simulink subsystem "adaptiveEcm"  (R2025b)
settings: Solver=VariableStepAuto  StartTime=0.0  StopTime=10.0  RelTol=1e-3
values from neighbouring files (symbols this model uses):
  ECM = ecmParams(TempDep=false, Degradation=false, IC=struct("soc0", zD(1, :), "T0C", mean(tC(1, :))))    [checkFastPlant.m]
undefined symbols (not defined in the file or in its folder): diff, trace
(part 1 of 2)
settings Model: Creator=SC-Br  LastModifiedBy=SC-Br

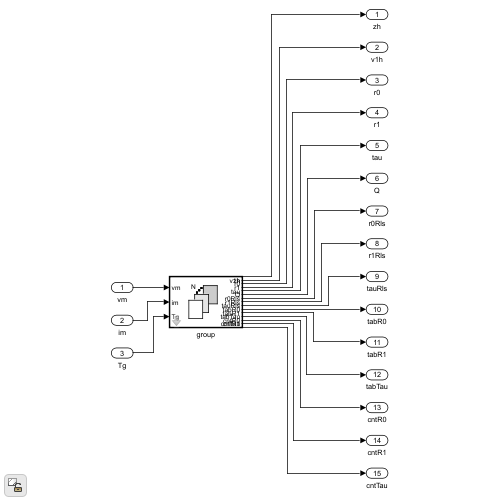
[thumbnail: Simulink's stored preview of the top-level diagram]
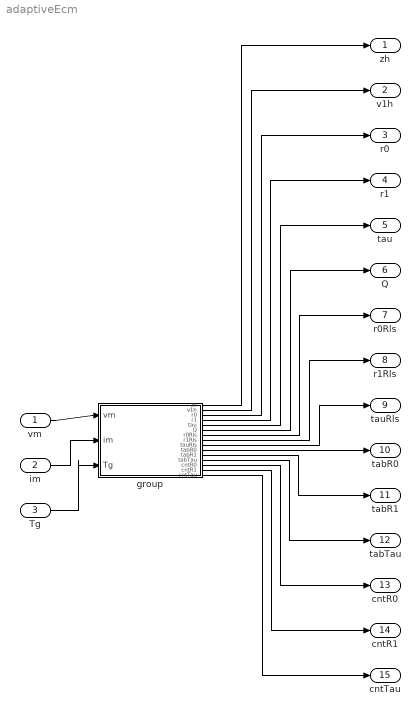
== system adaptiveEcm ==
  vm : Inport
  im : Inport  Port=2
  Tg : Inport  Port=3
  group : Subsystem  TreatAsAtomicUnit=on  mask{r0Init=ECM.est.init.r0, r1Init=ECM.est.init.r1, tauInit=ECM.est.init.tau, c0Init=ECM.est.init.count(:,:,:,1), c1Init=ECM.est.init.count(:,:,:,2), c2Init=ECM.est.init.count(:,:,:,3), QInit=ECM.est.init.Q, th0Init=ECM.est.init.th0, thRcInit=ECM.est.init.thRc, phiInit=ECM.est.init.phi}
  zh : Outport
  v1h : Outport  Port=2
  r0 : Outport  Port=3
  r1 : Outport  Port=4
  tau : Outport  Port=5
  Q : Outport  Port=6
  r0Rls : Outport  Port=7
  r1Rls : Outport  Port=8
  tauRls : Outport  Port=9
  tabR0 : Outport  Port=10
  tabR1 : Outport  Port=11
  tabTau : Outport  Port=12
  cntR0 : Outport  Port=13
  cntR1 : Outport  Port=14
  cntTau : Outport  Port=15
  wires:
  Tg/1 -> group/3(Tg)
  vm/1 -> group/1(vm)
  im/1 -> group/2(im)
  group/5(tau) -> tau/1
  group/12(tabTau) -> tabTau/1
  group/4(r1) -> r1/1
  group/11(tabR1) -> tabR1/1
  group/3(r0) -> r0/1
  group/10(tabR0) -> tabR0/1
  group/2(v1h) -> v1h/1
  group/9(tauRls) -> tauRls/1
  group/1(zh) -> zh/1
  group/6(Q) -> Q/1
  group/7(r0Rls) -> r0Rls/1
  group/8(r1Rls) -> r1Rls/1
  group/13(cntR0) -> cntR0/1
  group/14(cntR1) -> cntR1/1
  group/15(cntTau) -> cntTau/1

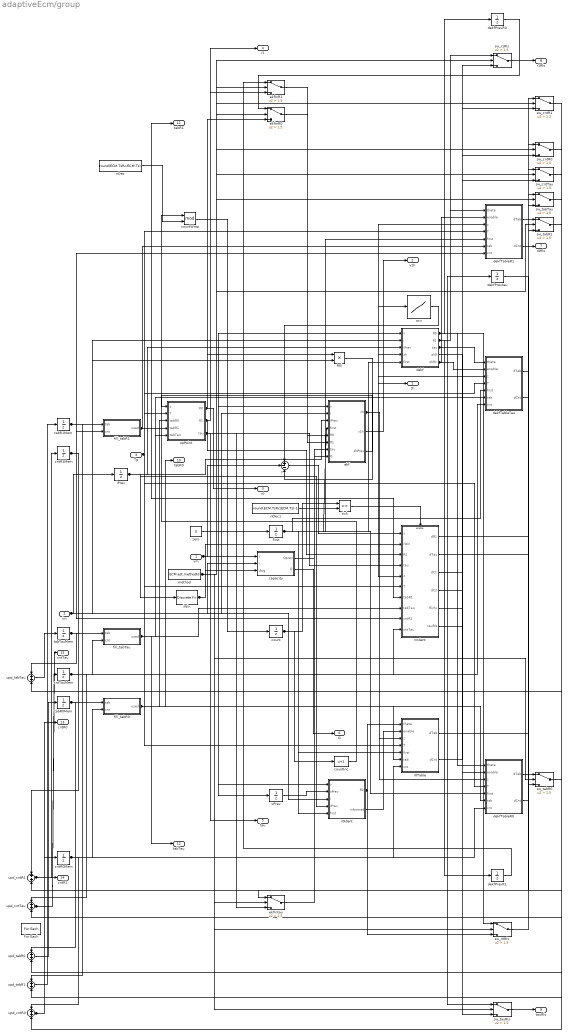
== system adaptiveEcm/group ==
  vm : Inport  PortDimensions=1  Partition=on  PartitionDimension=1  PartitionWidth=1  PartitionOffset=0
  im : Inport  Port=2  PortDimensions=1
  Tg : Inport  Port=3  PortDimensions=1  Partition=on  PartitionDimension=1  PartitionWidth=1  PartitionOffset=0
  For Each : ForEach  DisableCoverage=on  IterateSubsysMaskParameter=on,on,on,on,on,on,on,on,on,on  SubsysMaskParameterIterationDimension=3,3,3,3,3,3,2,2,2,2  SubsysMaskParameterIterationStepSize=1,1,1,1,1,1,1,1,1,1
  R0i : Product
  capacity : Subsystem
  cntR0Mem : UnitDelay  InitialCondition=c0Init  SampleTime=ECM.Ts  HasFrameUpgradeWarning=on
  cntR1Mem : UnitDelay  InitialCondition=c1Init  SampleTime=ECM.Ts  HasFrameUpgradeWarning=on
  cntTauMem : UnitDelay  InitialCondition=c2Init  SampleTime=ECM.Ts  HasFrameUpgradeWarning=on
  count : UnitDelay  SampleTime=ECM.Ts  HasFrameUpgradeWarning=on
  countInc : Bias  Bias=1  SaturateOnIntegerOverflow=off
  countWrap : Math  Operator=mod
  dekf : Subsystem
  dekfPrevR0 : UnitDelay  InitialCondition=exp(phiInit(1))  SampleTime=ECM.Ts  HasFrameUpgradeWarning=on
  dekfPrevR1 : UnitDelay  InitialCondition=exp(phiInit(2))  SampleTime=ECM.Ts  HasFrameUpgradeWarning=on
  dekfPrevtau : UnitDelay  InitialCondition=exp(phiInit(3))  SampleTime=ECM.Ts  HasFrameUpgradeWarning=on
  dekfTableR0 : Subsystem
  dekfTableR1 : Subsystem
  dekfTableTau : Subsystem
  ekf : Subsystem
  ekfInR0 : Switch  Criteria=u2 > Threshold  Threshold=1.5  SaturateOnIntegerOverflow=off  InputSameDT=off
  ekfInR1 : Switch  Criteria=u2 > Threshold  Threshold=1.5  SaturateOnIntegerOverflow=off  InputSameDT=off
  ekfIntau : Switch  Criteria=u2 > Threshold  Threshold=1.5  SaturateOnIntegerOverflow=off  InputSameDT=off
  fill_tabR0 : Subsystem
  fill_tabR1 : Subsystem
  fill_tabTau : Subsystem
  first : UnitDelay  InitialCondition=1  SampleTime=ECM.Ts  HasFrameUpgradeWarning=on
  iPrev : UnitDelay  SampleTime=ECM.Ts  HasFrameUpgradeWarning=on
  iWin : DiscreteFir  Coefficients=ones(1,round(ECM.TsRc/ECM.Ts))/round(ECM.TsRc/ECM.Ts)  SampleTime=ECM.Ts
  method : Constant  Value=ECM.est.methodId
  nDec : Constant  Value=round(ECM.TsRc/ECM.Ts)
  nDec1 : Constant  Value=round(ECM.TsRc/ECM.Ts)-1
  ocv : Lookup_n-D  NumberOfTableDimensions=1  BreakpointsForDimension1=ECM.est.socBp  Table=ECM.est.ocv  ExtrapMethod=Clip  UseLastTableValue=on  InternalRulePriority=Speed  RndMeth=Simplest
  opPoint : Subsystem
  r0Ident : Subsystem
  r0Table : Subsystem
  rcIdent : Subsystem  TreatAsAtomicUnit=on
  sw_cntR0 : Switch  Criteria=u2 > Threshold  Threshold=1.5  SaturateOnIntegerOverflow=off  InputSameDT=off
  sw_cntR1 : Switch  Criteria=u2 > Threshold  Threshold=1.5  SaturateOnIntegerOverflow=off  InputSameDT=off
  sw_cntTau : Switch  Criteria=u2 > Threshold  Threshold=1.5  SaturateOnIntegerOverflow=off  InputSameDT=off
  sw_r0Rls : Switch  Criteria=u2 > Threshold  Threshold=1.5  SaturateOnIntegerOverflow=off  InputSameDT=off
  sw_r1Rls : Switch  Criteria=u2 > Threshold  Threshold=1.5  SaturateOnIntegerOverflow=off  InputSameDT=off
  sw_tabR0 : Switch  Criteria=u2 > Threshold  Threshold=1.5  SaturateOnIntegerOverflow=off  InputSameDT=off
  sw_tabR1 : Switch  Criteria=u2 > Threshold  Threshold=1.5  SaturateOnIntegerOverflow=off  InputSameDT=off
  sw_tabTau : Switch  Criteria=u2 > Threshold  Threshold=1.5  SaturateOnIntegerOverflow=off  InputSameDT=off
  sw_tauRls : Switch  Criteria=u2 > Threshold  Threshold=1.5  SaturateOnIntegerOverflow=off  InputSameDT=off
  tabR0Mem : UnitDelay  InitialCondition=r0Init  SampleTime=ECM.Ts  HasFrameUpgradeWarning=on
  tabR1Mem : UnitDelay  InitialCondition=r1Init  SampleTime=ECM.Ts  HasFrameUpgradeWarning=on
  tabTauMem : UnitDelay  InitialCondition=tauInit  SampleTime=ECM.Ts  HasFrameUpgradeWarning=on
  tick : RelationalOperator  Operator===  OutDataTypeStr=boolean  RndMeth=Simplest  InputSameDT=off
  upd_cntR0 : Sum
  upd_cntR1 : Sum
  upd_cntTau : Sum
  upd_tabR0 : Sum
  upd_tabR1 : Sum
  upd_tabTau : Sum
  vPrev : UnitDelay  SampleTime=ECM.Ts  HasFrameUpgradeWarning=on
  y : Sum  Inputs=+--
  zero : Constant  Value=0
  zh : Outport  ConcatenationDimension=1
  v1h : Outport  Port=2  ConcatenationDimension=1
  r0 : Outport  Port=3  ConcatenationDimension=1
  r1 : Outport  Port=4  ConcatenationDimension=1
  tau : Outport  Port=5  ConcatenationDimension=1
  Q : Outport  Port=6  ConcatenationDimension=1
  r0Rls : Outport  Port=7  ConcatenationDimension=1
  r1Rls : Outport  Port=8  ConcatenationDimension=1
  tauRls : Outport  Port=9  ConcatenationDimension=1
  tabR0 : Outport  Port=10  ConcatenationDimension=3
  tabR1 : Outport  Port=11  ConcatenationDimension=3
  tabTau : Outport  Port=12  ConcatenationDimension=3
  cntR0 : Outport  Port=13  ConcatenationDimension=3
  cntR1 : Outport  Port=14  ConcatenationDimension=3
  cntTau : Outport  Port=15  ConcatenationDimension=3
  wires:
  upd_cntR0/1 -> cntR0Mem/1, cntR0/1
  tabR1Mem/1 -> upd_tabR1/1, fill_tabR1/1(tab)
  dekf/1(R0) -> dekfTableR0/1(theta), dekfPrevR0/1, sw_r0Rls/1
  fill_tabTau/1(used) -> dekfTableTau/6(tab), tabTau/1, rcIdent/8(tabTau), opPoint/5(tabTau)
  sw_tauRls/1 -> tauRls/1
  rcIdent/6(tauRls) -> sw_tauRls/3
  sw_r1Rls/1 -> r1Rls/1
  vm/1 -> ekf/1(v), r0Ident/1(v), dekf/1(v), vPrev/1, y/2, capacity/1(v)
  dekfPrevtau/1 -> ekfIntau/1
  zero/1 -> first/1
  nDec/1 -> countWrap/2
  sw_r0Rls/1 -> r0Rls/1
  r0Ident/2(informed) -> r0Table/2(enable)
  fill_tabR0/1(used) -> dekfTableR0/6(tab), r0Table/6(tab), opPoint/3(tabR0), tabR0/1
  dekfTableR1/1(dTab) -> sw_tabR1/1
  capacity/2(Q) -> Q/1
  rcIdent/5(R1rls) -> sw_r1Rls/3
  ekf/2(v1h) -> v1h/1
  fill_tabR1/1(used) -> dekfTableR1/6(tab), rcIdent/7(tabR1), opPoint/4(tabR1), tabR1/1
  ekfInR1/1 -> ekf/6(R1)
  rcIdent/4(dC2) -> sw_cntTau/3
  dekf/4(ok0) -> dekfTableR0/2(enable)
  dekfTableR0/1(dTab) -> sw_tabR0/1
  im/1 -> capacity/2(i), dekf/2(i), R0i/2, r0Ident/3(i), ekf/2(i), iPrev/1
  dekfTableTau/2(dCnt) -> sw_cntTau/1
  upd_tabR0/1 -> tabR0Mem/1
  opPoint/1(R0) -> R0i/1, ekfInR0/3, r0/1
  sw_tabTau/1 -> upd_tabTau/2
  ekf/3(zhPrev) -> opPoint/1(z)
  ekfInR0/1 -> ekf/5(R0)
  opPoint/2(R1) -> rcIdent/3(R1), r1/1, ekfInR1/3
  ekf/1(zh) -> dekfTableTau/3(z), dekfTableR1/3(z), dekfTableR0/3(z), ocv/1, rcIdent/5(z), dekf/4(zh), zh/1, r0Table/3(z)
  dekfTableTau/1(dTab) -> sw_tabTau/1
  cntR1Mem/1 -> upd_cntR1/1, rcIdent/9(cntR1), dekfTableR1/7(cnt), fill_tabR1/2(cnt)
  iWin/1 -> rcIdent/2(iWin), capacity/3(iAvg)
  dekfTableR1/2(dCnt) -> sw_cntR1/1
  rcIdent/3(dC1) -> sw_cntR1/3
  cntTauMem/1 -> upd_cntTau/1, rcIdent/10(cntTau), dekfTableTau/7(cnt), fill_tabTau/2(cnt)
  rcIdent/1(dR1) -> sw_tabR1/3
  r0Ident/1(R0) -> sw_r0Rls/3, r0Table/1(theta)
  first/1 -> dekfTableR1/5(first), dekfTableTau/5(first), dekfTableR0/5(first), dekf/5(first), r0Ident/5(first), r0Table/5(first), ekf/4(first)
  sw_tabR1/1 -> upd_tabR1/2
  opPoint/3(tau) -> rcIdent/4(tau), tau/1, ekfIntau/3
  dekfTableR0/2(dCnt) -> sw_cntR0/1
  countWrap/1 -> count/1
  dekf/3(tau) -> dekfTableTau/1(theta), sw_tauRls/1, dekfPrevtau/1
  upd_cntTau/1 -> cntTauMem/1, cntTau/1
  Tg/1 -> dekfTableR0/4(T), dekfTableTau/4(T), dekfTableR1/4(T), rcIdent/6(T), opPoint/2(T), r0Table/4(T)
  capacity/1(Qprev) -> ekf/8(Q)
  ekfIntau/1 -> ekf/7(tau)
  vPrev/1 -> r0Ident/2(vPrev)
  method/1 -> sw_tabR0/2, sw_tabR1/2, sw_cntR1/2, sw_tabTau/2, sw_r1Rls/2, sw_tauRls/2, sw_r0Rls/2, sw_cntTau/2, ekfInR1/2, ekfIntau/2, sw_cntR0/2, ekfInR0/2
  nDec1/1 -> tick/2
  iPrev/1 -> r0Ident/4(iPrev), ekf/3(iPrev), dekf/3(iPrev), iWin/1
  upd_tabTau/1 -> tabTauMem/1
  upd_cntR1/1 -> cntR1Mem/1, cntR1/1
  r0Table/1(dTab) -> sw_tabR0/3
  dekfPrevR0/1 -> ekfInR0/1
  upd_tabR1/1 -> tabR1Mem/1
  dekf/5(okRc) -> dekfTableR1/2(enable), dekfTableTau/2(enable)
  dekf/2(R1) -> dekfTableR1/1(theta), dekfPrevR1/1, sw_r1Rls/1
  count/1 -> countInc/1, tick/1
  tabTauMem/1 -> upd_tabTau/1, fill_tabTau/1(tab)
  cntR0Mem/1 -> upd_cntR0/1, r0Table/7(cnt), dekfTableR0/7(cnt), fill_tabR0/2(cnt)
  sw_cntR0/1 -> upd_cntR0/2
  tabR0Mem/1 -> upd_tabR0/1, fill_tabR0/1(tab)
  y/1 -> rcIdent/1(y)
  r0Table/2(dCnt) -> sw_cntR0/3
  rcIdent/2(dTau) -> sw_tabTau/3
  tick/1 -> rcIdent/Enable
  R0i/1 -> y/3
  countInc/1 -> countWrap/1
  sw_tabR0/1 -> upd_tabR0/2
  dekfPrevR1/1 -> ekfInR1/1
  ocv/1 -> y/1
  sw_cntR1/1 -> upd_cntR1/2
  sw_cntTau/1 -> upd_cntTau/2

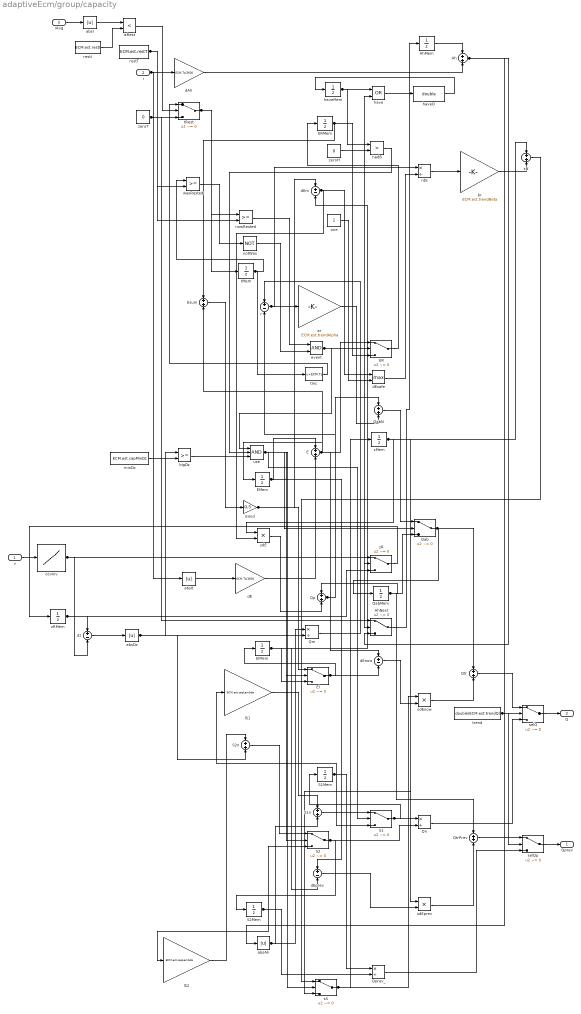
== system adaptiveEcm/group/capacity ==
  v : Inport  PortDimensions=1
  i : Inport  Port=2  PortDimensions=1
  iAvg : Inport  Port=3  PortDimensions=1
  Ah : Sum
  AhMem : UnitDelay  SampleTime=ECM.Ts  HasFrameUpgradeWarning=on
  AhNext : Switch  Criteria=u2 ~= 0  SaturateOnIntegerOverflow=off  InputSameDT=off
  E : Sum
  EMem : UnitDelay  SampleTime=ECM.Ts  HasFrameUpgradeWarning=on
  ER : Switch  Criteria=u2 ~= 0  SaturateOnIntegerOverflow=off  InputSameDT=off
  ERMem : UnitDelay  SampleTime=ECM.Ts  HasFrameUpgradeWarning=on
  El : Switch  Criteria=u2 ~= 0  SaturateOnIntegerOverflow=off  InputSameDT=off
  ElMem : UnitDelay  SampleTime=ECM.Ts  HasFrameUpgradeWarning=on
  Emid : Gain  Gain=0.5
  Esum : Sum
  Qab : Switch  Criteria=u2 ~= 0  SaturateOnIntegerOverflow=off  InputSameDT=off
  QabMem : UnitDelay  InitialCondition=QInit  SampleTime=ECM.Ts  HasFrameUpgradeWarning=on
  QabN : Sum
  Qm : Product  Inputs=*/
  Qn : Product  Inputs=*/
  Qp : Sum
  Qprev_ : Product  Inputs=*/
  Qtr : Sum
  QtrPrev : Sum
  S1 : Switch  Criteria=u2 ~= 0  SaturateOnIntegerOverflow=off  InputSameDT=off
  S1Mem : UnitDelay  InitialCondition=ECM.est.capW0*QInit  SampleTime=ECM.Ts  HasFrameUpgradeWarning=on
  S1n : Sum
  S2 : Switch  Criteria=u2 ~= 0  SaturateOnIntegerOverflow=off  InputSameDT=off
  S2Mem : UnitDelay  InitialCondition=ECM.est.capW0  SampleTime=ECM.Ts  HasFrameUpgradeWarning=on
  S2n : Sum
  absAh : Abs  SaturateOnIntegerOverflow=off
  absDz : Abs  SaturateOnIntegerOverflow=off
  absI : Abs  SaturateOnIntegerOverflow=off
  absIt : Abs  SaturateOnIntegerOverflow=off
  ar : Gain  Gain=ECM.est.trendAlpha
  bigDz : RelationalOperator  OutDataTypeStr=boolean  RndMeth=Simplest  InputSameDT=off
  br : Gain  Gain=ECM.est.trendBeta
  dAh : Gain  Gain=ECM.Ts/3600
  dE : Gain  Gain=ECM.Ts/3600
  dEm : Sum  Inputs=+-
  dEnow : Sum  Inputs=+-
  dEprev : Sum  Inputs=+-
  dEsafe : MinMax  Function=max  Inputs=2
  dz : Sum  Inputs=+-
  event : Logic  AllPortsSameDT=off  OutDataTypeStr=boolean
  hadB : RelationalOperator  Operator=>  OutDataTypeStr=boolean  RndMeth=Simplest  InputSameDT=off
  have : Logic  Operator=OR  AllPortsSameDT=off  OutDataTypeStr=boolean
  haveD : DataTypeConversion  OutDataTypeStr=double  SaturateOnIntegerOverflow=off  RndMeth=Floor
  haveMem : UnitDelay  SampleTime=ECM.Ts  HasFrameUpgradeWarning=on
  isRest : RelationalOperator  Operator=<  OutDataTypeStr=boolean  RndMeth=Simplest  InputSameDT=off
  lS1 : Gain  Gain=ECM.est.capLambda
  lS2 : Gain  Gain=ECM.est.capLambda
  minDz : Constant  Value=ECM.est.capMinDz
  notWas : Logic  Operator=NOT  AllPortsSameDT=off  OutDataTypeStr=boolean
  nowRested : RelationalOperator  OutDataTypeStr=boolean  RndMeth=Simplest  InputSameDT=off
  ocvInv : Lookup_n-D  NumberOfTableDimensions=1  BreakpointsForDimension1=ECM.est.ocv  Table=ECM.est.socBp  ExtrapMethod=Clip  UseLastTableValue=on  InternalRulePriority=Speed  RndMeth=Simplest
  one : Constant
  r : Sum  Inputs=+-
  rdE : Product  Inputs=*/
  restI : Constant  Value=ECM.est.restI
  restT : Constant  Value=ECM.est.restT
  sMem : UnitDelay  SampleTime=ECM.Ts  HasFrameUpgradeWarning=on
  sN : Sum
  sS : Switch  Criteria=u2 ~= 0  SaturateOnIntegerOverflow=off  InputSameDT=off
  sdE : Product
  sdEnow : Product
  sdEprev : Product
  selQ : Switch  Criteria=u2 ~= 0  SaturateOnIntegerOverflow=off  InputSameDT=off
  selQp : Switch  Criteria=u2 ~= 0  SaturateOnIntegerOverflow=off  InputSameDT=off
  tInc : Bias  Bias=ECM.Ts  SaturateOnIntegerOverflow=off
  tMem : UnitDelay  SampleTime=ECM.Ts  HasFrameUpgradeWarning=on
  tRest : Switch  Criteria=u2 ~= 0  SaturateOnIntegerOverflow=off  InputSameDT=off
  trend : Constant  Value=double(ECM.est.trendQ)
  use : Logic  Inputs=3  AllPortsSameDT=off  OutDataTypeStr=boolean
  wasRested : RelationalOperator  OutDataTypeStr=boolean  RndMeth=Simplest  InputSameDT=off
  zR : Switch  Criteria=u2 ~= 0  SaturateOnIntegerOverflow=off  InputSameDT=off
  zRMem : UnitDelay  SampleTime=ECM.Ts  HasFrameUpgradeWarning=on
  zeroH : Constant  Value=0
  zeroT : Constant  Value=0
  Qprev : Outport
  Q : Outport  Port=2
  wires:
  ERMem/1 -> Esum/1, ER/3
  absIt/1 -> dE/1
  v/1 -> ocvInv/1
  isRest/1 -> tRest/2
  ar/1 -> QabN/2
  wasRested/1 -> notWas/1
  restI/1 -> isRest/2
  event/1 -> use/1, have/2, AhNext/2, ER/2, zR/2
  iAvg/1 -> absI/1
  S2Mem/1 -> lS2/1, Qprev_/2, S2/3
  zRMem/1 -> dz/1, zR/3
  restT/1 -> nowRested/2, wasRested/2
  ocvInv/1 -> dz/2, zR/1
  absI/1 -> isRest/1
  dz/1 -> absDz/1
  i/1 -> absIt/1, dAh/1
  dEnow/1 -> sdEnow/2
  zeroT/1 -> AhNext/1, tRest/3
  nowRested/1 -> event/1
  minDz/1 -> bigDz/2
  absDz/1 -> Qm/2, S2n/2, bigDz/1
  dAh/1 -> Ah/2
  zR/1 -> zRMem/1
  tRest/1 -> tMem/1, nowRested/1
  one/1 -> dEsafe/2
  Esum/1 -> Emid/1
  bigDz/1 -> use/3
  lS2/1 -> S2n/1
  notWas/1 -> event/2
  zeroH/1 -> hadB/2
  tMem/1 -> tInc/1, wasRested/1
  r/1 -> rdE/1, ar/1
  use/1 -> S1/2, S2/2, Qab/2, El/2, sS/2
  tInc/1 -> tRest/1
  EMem/1 -> E/1, dEprev/1
  S2/1 -> S2Mem/1, Qn/2
  Emid/1 -> dEm/1, El/1
  sdE/1 -> Qp/2
  dE/1 -> E/2
  dEprev/1 -> sdEprev/2
  ElMem/1 -> dEm/2, El/3, dEprev/2
  lS1/1 -> S1n/1
  S2n/1 -> S2/1
  absAh/1 -> S1n/2, Qm/1
  haveMem/1 -> have/1, hadB/1
  dEm/1 -> sdE/2, dEsafe/1
  E/1 -> EMem/1, Esum/2, dEnow/1, ER/1
  dEsafe/1 -> rdE/2
  Qp/1 -> r/2, QabN/1
  AhMem/1 -> Ah/1
  have/1 -> haveD/1
  sS/1 -> sdEnow/1, sMem/1
  Qm/1 -> r/1
  El/1 -> ElMem/1, dEnow/2
  S1Mem/1 -> lS1/1, Qprev_/1, S1/3
  AhNext/1 -> AhMem/1
  Qprev_/1 -> selQp/3
  S1n/1 -> S1/1
  hadB/1 -> use/2
  ER/1 -> ERMem/1
  QabN/1 -> Qab/1
  sMem/1 -> sdE/1, sN/1, sdEprev/1, sS/3
  S1/1 -> S1Mem/1, Qn/1
  QabMem/1 -> Qp/1, QtrPrev/1, Qab/3
  haveD/1 -> haveMem/1
  rdE/1 -> br/1
  Qab/1 -> QabMem/1, Qtr/1
  sdEnow/1 -> Qtr/2
  Qn/1 -> selQ/3
  sdEprev/1 -> QtrPrev/2
  Ah/1 -> absAh/1, AhNext/3
  br/1 -> sN/2
  Qtr/1 -> selQ/1
  trend/1 -> selQ/2, selQp/2
  QtrPrev/1 -> selQp/1
  sN/1 -> sS/1
  selQ/1 -> Q/1
  selQp/1 -> Qprev/1

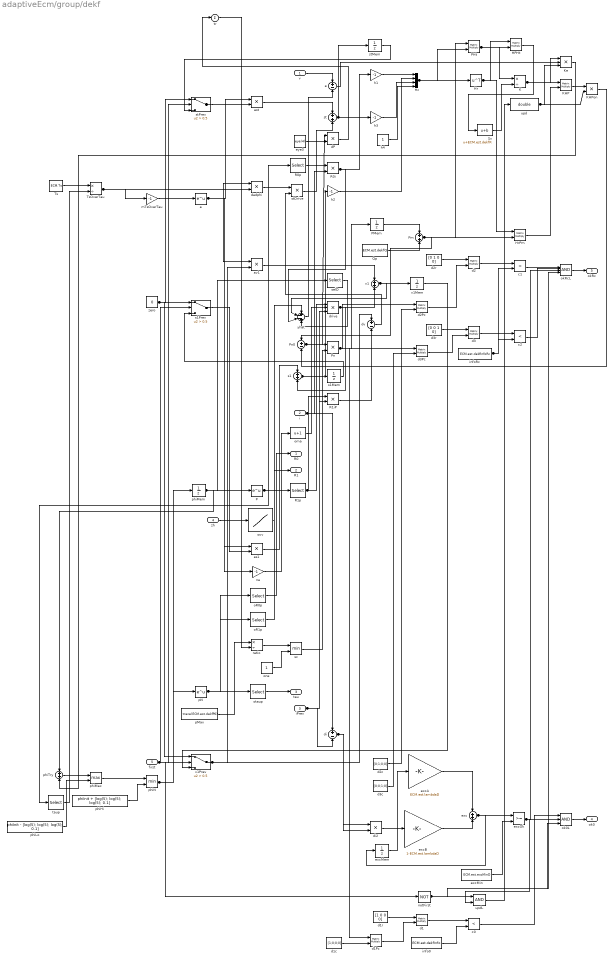
== system adaptiveEcm/group/dekf ==
  v : Inport  PortDimensions=1
  i : Inport  Port=2  PortDimensions=1
  iPrev : Inport  Port=3  PortDimensions=1
  zh : Inport  Port=4  PortDimensions=1
  first : Inport  Port=5  PortDimensions=1
  HPHt : Product  Multiplication=Matrix(*)
  Hc : Concatenate  NumInputs=4  Mode=Multidimensional array
  Hr : Math  Operator=transpose
  HrPm : Product  Multiplication=Matrix(*)
  K : Product  Inputs=*/
  KHP : Product  Multiplication=Matrix(*)
  KHPon : Product
  Ke : Product  Inputs=3
  PHt : Product  Multiplication=Matrix(*)
  PMem : UnitDelay  InitialCondition=ECM.est.dekfP0  SampleTime=ECM.Ts  HasFrameUpgradeWarning=on
  Pm : Sum
  Pn : Product
  Pn0 : Sum  Inputs=+-
  Qp : Constant  Value=ECM.est.dekfQ
  R0i : Product
  R0p : Selector  InputPortWidth=4  IndexOptions=Index vector (dialog)  Indices=1  OutputSizes=1
  R1iP : Product
  R1p : Selector  InputPortWidth=4  IndexOptions=Index vector (dialog)  Indices=2  OutputSizes=1
  Sv : Bias  Bias=ECM.est.dekfR  SaturateOnIntegerOverflow=off
  Ts : Constant  Value=ECM.Ts
  TsOverTau : Product  Inputs=*/
  a : Math
  as1 : Product
  ast : Product
  av1 : Product
  c0 : RelationalOperator  Operator=<  OutDataTypeStr=boolean  RndMeth=Simplest  InputSameDT=off
  c1 : RelationalOperator  Operator=<  OutDataTypeStr=boolean  RndMeth=Simplest  InputSameDT=off
  c2 : RelationalOperator  Operator=<  OutDataTypeStr=boolean  RndMeth=Simplest  InputSameDT=off
  d1 : Product  Multiplication=Matrix(*)
  d1Pc : Product  Multiplication=Matrix(*)
  d1c : Constant  Value=[1;0;0;0]  VectorParams1D=off
  d1r : Constant  Value=[1 0 0 0]  VectorParams1D=off
  d2 : Product  Multiplication=Matrix(*)
  d2Pc : Product  Multiplication=Matrix(*)
  d2c : Constant  Value=[0;1;0;0]  VectorParams1D=off
  d2r : Constant  Value=[0 1 0 0]  VectorParams1D=off
  d3 : Product  Multiplication=Matrix(*)
  d3Pc : Product  Multiplication=Matrix(*)
  d3c : Constant  Value=[0;0;1;0]  VectorParams1D=off
  d3r : Constant  Value=[0 0 1 0]  VectorParams1D=off
  dP : Product
  dadphi : Product
  di : Sum  Inputs=+-
  di2 : Product
  drive : Product  Inputs=3
  dv : Sum  Inputs=+-
  e : Sum  Inputs=+-
  exc : Sum
  excA : Gain  Gain=ECM.est.lambdaD
  excB : Gain  Gain=1-ECM.est.lambdaD
  excMem : UnitDelay  SampleTime=ECM.Ts  HasFrameUpgradeWarning=on
  excMin : Constant  Value=ECM.est.excMinD
  excOk : RelationalOperator  OutDataTypeStr=boolean  RndMeth=Simplest  InputSameDT=off
  eye3 : Constant  Value=eye(4)
  h1 : Gain  Gain=-1
  h2 : Gain  Gain=-1
  h3 : Gain  Gain=-1
  h4 : Constant
  info0 : Constant  Value=ECM.est.dekfInfo
  infoRc : Constant  Value=ECM.est.dekfInfoRc
  mTsOverTau : Gain  Gain=-1
  na : Gain  Gain=-1
  notFirst : Logic  Operator=NOT  AllPortsSameDT=off  OutDataTypeStr=boolean
  oR0p : Selector  InputPortWidth=4  IndexOptions=Index vector (dialog)  Indices=1  OutputSizes=1
  oR1p : Selector  InputPortWidth=4  IndexOptions=Index vector (dialog)  Indices=2  OutputSizes=1
  ocv : Lookup_n-D  NumberOfTableDimensions=1  BreakpointsForDimension1=ECM.est.socBp  Table=ECM.est.ocv  ExtrapMethod=Clip  UseLastTableValue=on  InternalRulePriority=Speed  RndMeth=Simplest
  ok0L : Logic  Inputs=3  AllPortsSameDT=off  OutDataTypeStr=boolean
  okRcL : Logic  Inputs=4  AllPortsSameDT=off  OutDataTypeStr=boolean
  oma : Bias  Bias=1  SaturateOnIntegerOverflow=off
  one : Constant
  otaup : Selector  InputPortWidth=4  IndexOptions=Index vector (dialog)  Indices=3  OutputSizes=1
  p : Math
  pMax : Constant  Value=trace(ECM.est.dekfP0)
  pN : Math
  phiHi : Constant  Value=phiInit + [log(5); log(5); log(5); 0.1]
  phiLo : Constant  Value=phiInit - [log(5); log(5); log(5); 0.1]
  phiMax : MinMax  Function=max  Inputs=2
  phiMem : UnitDelay  InitialCondition=phiInit  SampleTime=ECM.Ts  HasFrameUpgradeWarning=on
  phiN : MinMax  Inputs=2
  phiTry : Sum
  ratio : Product  Inputs=*/
  s1 : Sum
  s1Mem : UnitDelay  SampleTime=ECM.Ts  HasFrameUpgradeWarning=on
  s1Prev : Switch  Criteria=u2 > Threshold  Threshold=0.5  SaturateOnIntegerOverflow=off  InputSameDT=off
  sc : MinMax  Inputs=2
  selD : Selector  InputPortWidth=4  IndexOptions=Index vector (dialog)  Indices=4  OutputSizes=1
  st : Sum
  stDrive : Product
  stMem : UnitDelay  SampleTime=ECM.Ts  HasFrameUpgradeWarning=on
  stPrev : Switch  Criteria=u2 > Threshold  Threshold=0.5  SaturateOnIntegerOverflow=off  InputSameDT=off
  taup : Selector  InputPortWidth=4  IndexOptions=Index vector (dialog)  Indices=3  OutputSizes=1
  tr : Sum  Inputs=+
  upd : DataTypeConversion  OutDataTypeStr=double  SaturateOnIntegerOverflow=off  RndMeth=Floor
  updL : Logic  AllPortsSameDT=off  OutDataTypeStr=boolean
  v1 : Sum
  v1Mem : UnitDelay  SampleTime=ECM.Ts  HasFrameUpgradeWarning=on
  v1Prev : Switch  Criteria=u2 > Threshold  Threshold=0.5  SaturateOnIntegerOverflow=off  InputSameDT=off
  yhat : Sum  Inputs=+--+
  zero : Constant  Value=0
  R0 : Outport
  R1 : Outport  Port=2
  tau : Outport  Port=3
  ok0 : Outport  Port=4
  okRc : Outport  Port=5
  wires:
  selD/1 -> yhat/4
  TsOverTau/1 -> mTsOverTau/1, dadphi/2
  Hr/1 -> HPHt/1, HrPm/1
  dP/1 -> tr/1
  oma/1 -> drive/2
  R0p/1 -> R0i/1
  Pn0/1 -> dP/1, Pn/1
  pMax/1 -> ratio/1
  Ts/1 -> TsOverTau/1
  phiHi/1 -> phiN/2
  phiLo/1 -> phiMax/2
  stMem/1 -> stPrev/3
  phiTry/1 -> phiMax/1
  mTsOverTau/1 -> a/1
  sc/1 -> Pn/2
  h1/1 -> Hc/1
  v1Prev/1 -> dv/1, av1/2
  taup/1 -> TsOverTau/2
  iPrev/1 -> di/2, drive/3, R1iP/2
  phiMax/1 -> phiN/1
  R1p/1 -> drive/1, R1iP/1
  eye3/1 -> dP/2
  zero/1 -> v1Prev/1, s1Prev/1, stPrev/1
  e/1 -> Ke/2
  upd/1 -> KHPon/2, Ke/3
  first/1 -> v1Prev/2, s1Prev/2, stPrev/2, notFirst/1
  s1Mem/1 -> s1Prev/3
  R0i/1 -> yhat/3, h1/1
  phiN/1 -> phiMem/1, pN/1
  tr/1 -> ratio/2
  stPrev/1 -> ast/2
  s1Prev/1 -> as1/2
  a/1 -> av1/1, dadphi/1, na/1, ast/1, as1/1
  R1iP/1 -> dv/2
  phiMem/1 -> phiTry/1, selD/1, p/1
  zh/1 -> ocv/1
  pN/1 -> oR0p/1, otaup/1, oR1p/1
  ast/1 -> st/1
  stDrive/1 -> st/2
  dadphi/1 -> stDrive/1
  v1/1 -> yhat/2, v1Mem/1
  av1/1 -> v1/1
  h4/1 -> Hc/4
  p/1 -> taup/1, R0p/1, R1p/1
  di/1 -> di2/1, di2/2
  ocv/1 -> yhat/1
  yhat/1 -> e/2
  as1/1 -> s1/1
  na/1 -> oma/1
  oR0p/1 -> R0/1
  Pn/1 -> d3Pc/1, PMem/1, d1Pc/1, d2Pc/1
  drive/1 -> s1/2, v1/2
  oR1p/1 -> R1/1
  ratio/1 -> sc/1
  one/1 -> sc/2
  otaup/1 -> tau/1
  v/1 -> e/1
  s1/1 -> s1Mem/1, h2/1
  i/1 -> di/1, R0i/2
  st/1 -> stMem/1, h3/1
  h2/1 -> Hc/2
  d1c/1 -> d1Pc/2
  h3/1 -> Hc/3
  PMem/1 -> Pm/1
  Qp/1 -> Pm/2
  dv/1 -> stDrive/2
  d2c/1 -> d2Pc/2
  d3c/1 -> d3Pc/2
  di2/1 -> excB/1
  excMem/1 -> excA/1
  d1r/1 -> d1/1
  d1Pc/1 -> d1/2
  Hc/1 -> Hr/1, PHt/2
  Pm/1 -> Pn0/1, PHt/1, HrPm/2
  d2r/1 -> d2/1
  v1Mem/1 -> v1Prev/3
  d2Pc/1 -> d2/2
  d3r/1 -> d3/1
  d3Pc/1 -> d3/2
  excA/1 -> exc/1
  excB/1 -> exc/2
  notFirst/1 -> okRcL/4, updL/1, ok0L/3
  d1/1 -> c0/1
  info0/1 -> c0/2
  PHt/1 -> K/1, HPHt/2
  Sv/1 -> K/2
  d2/1 -> c1/1
  d3/1 -> c2/1
  infoRc/1 -> c1/2, c2/2
  exc/1 -> excOk/1, excMem/1
  excMin/1 -> excOk/2
  updL/1 -> upd/1
  c0/1 -> ok0L/1
  HPHt/1 -> Sv/1
  K/1 -> Ke/1, KHP/1
  HrPm/1 -> KHP/2
  c1/1 -> okRcL/1
  c2/1 -> okRcL/2
  excOk/1 -> updL/2, okRcL/3, ok0L/2
  Ke/1 -> phiTry/2
  KHP/1 -> KHPon/1
  okRcL/1 -> okRc/1
  ok0L/1 -> ok0/1
  KHPon/1 -> Pn0/2

== system adaptiveEcm/group/dekfTableR0 ==
  theta : Inport  PortDimensions=1
  enable : Inport  Port=2  PortDimensions=1
  z : Inport  Port=3  PortDimensions=1
  T : Inport  Port=4  PortDimensions=1
  first : Inport  Port=5  PortDimensions=1
  tab : Inport  Port=6  PortDimensions=[numel(ECM.est.socBp) numel(ECM.est.tBpC)]
  cnt : Inport  Port=7  PortDimensions=[numel(ECM.est.socBp) numel(ECM.est.tBpC)]
  TLag : Sum
  TLagA : Gain  Gain=ECM.est.lambdaD
  TLagB : Gain  Gain=1-ECM.est.lambdaD
  TLagMem : UnitDelay  SampleTime=-1  HasFrameUpgradeWarning=on
  TLagOld : Switch  Criteria=u2 > Threshold  Threshold=0.5  SaturateOnIntegerOverflow=off  InputSameDT=off
  nodeUpdate : Subsystem
  zLag : Sum
  zLagA : Gain  Gain=ECM.est.lambdaD
  zLagB : Gain  Gain=1-ECM.est.lambdaD
  zLagMem : UnitDelay  SampleTime=-1  HasFrameUpgradeWarning=on
  zLagOld : Switch  Criteria=u2 > Threshold  Threshold=0.5  SaturateOnIntegerOverflow=off  InputSameDT=off
  dTab : Outport
  dCnt : Outport  Port=2
  wires:
  z/1 -> zLagB/1, zLagOld/1
  TLagOld/1 -> TLagA/1
  TLagMem/1 -> TLagOld/3
  zLagA/1 -> zLag/1
  zLagB/1 -> zLag/2
  T/1 -> TLagOld/1, TLagB/1
  first/1 -> TLagOld/2, zLagOld/2
  zLagOld/1 -> zLagA/1
  TLag/1 -> TLagMem/1, nodeUpdate/4(T)
  TLagB/1 -> TLag/2
  TLagA/1 -> TLag/1
  theta/1 -> nodeUpdate/1(theta)
  zLag/1 -> zLagMem/1, nodeUpdate/3(z)
  enable/1 -> nodeUpdate/2(enable)
  zLagMem/1 -> zLagOld/3
  tab/1 -> nodeUpdate/5(tab)
  cnt/1 -> nodeUpdate/6(cnt)
  nodeUpdate/1(dTab) -> dTab/1
  nodeUpdate/2(dCnt) -> dCnt/1

== system adaptiveEcm/group/dekfTableR1 ==
  theta : Inport  PortDimensions=1
  enable : Inport  Port=2  PortDimensions=1
  z : Inport  Port=3  PortDimensions=1
  T : Inport  Port=4  PortDimensions=1
  first : Inport  Port=5  PortDimensions=1
  tab : Inport  Port=6  PortDimensions=[numel(ECM.est.socBp) numel(ECM.est.tBpC)]
  cnt : Inport  Port=7  PortDimensions=[numel(ECM.est.socBp) numel(ECM.est.tBpC)]
  TLag : Sum
  TLagA : Gain  Gain=ECM.est.lambdaD
  TLagB : Gain  Gain=1-ECM.est.lambdaD
  TLagMem : UnitDelay  SampleTime=-1  HasFrameUpgradeWarning=on
  TLagOld : Switch  Criteria=u2 > Threshold  Threshold=0.5  SaturateOnIntegerOverflow=off  InputSameDT=off
  nodeUpdate : Subsystem
  zLag : Sum
  zLagA : Gain  Gain=ECM.est.lambdaD
  zLagB : Gain  Gain=1-ECM.est.lambdaD
  zLagMem : UnitDelay  SampleTime=-1  HasFrameUpgradeWarning=on
  zLagOld : Switch  Criteria=u2 > Threshold  Threshold=0.5  SaturateOnIntegerOverflow=off  InputSameDT=off
  dTab : Outport
  dCnt : Outport  Port=2
  wires:
  z/1 -> zLagOld/1, zLagB/1
  first/1 -> zLagOld/2, TLagOld/2
  TLagOld/1 -> TLagA/1
  T/1 -> TLagB/1, TLagOld/1
  zLagA/1 -> zLag/1
  zLagB/1 -> zLag/2
  zLagOld/1 -> zLagA/1
  TLagA/1 -> TLag/1
  TLagB/1 -> TLag/2
  nodeUpdate/1(dTab) -> dTab/1
  theta/1 -> nodeUpdate/1(theta)
  zLag/1 -> zLagMem/1, nodeUpdate/3(z)
  enable/1 -> nodeUpdate/2(enable)
  tab/1 -> nodeUpdate/5(tab)
  TLag/1 -> nodeUpdate/4(T), TLagMem/1
  cnt/1 -> nodeUpdate/6(cnt)
  zLagMem/1 -> zLagOld/3
  nodeUpdate/2(dCnt) -> dCnt/1
  TLagMem/1 -> TLagOld/3

== system adaptiveEcm/group/dekfTableTau ==
  theta : Inport  PortDimensions=1
  enable : Inport  Port=2  PortDimensions=1
  z : Inport  Port=3  PortDimensions=1
  T : Inport  Port=4  PortDimensions=1
  first : Inport  Port=5  PortDimensions=1
  tab : Inport  Port=6  PortDimensions=[numel(ECM.est.socBp) numel(ECM.est.tBpC)]
  cnt : Inport  Port=7  PortDimensions=[numel(ECM.est.socBp) numel(ECM.est.tBpC)]
  TLag : Sum
  TLagA : Gain  Gain=ECM.est.lambdaD
  TLagB : Gain  Gain=1-ECM.est.lambdaD
  TLagMem : UnitDelay  SampleTime=-1  HasFrameUpgradeWarning=on
  TLagOld : Switch  Criteria=u2 > Threshold  Threshold=0.5  SaturateOnIntegerOverflow=off  InputSameDT=off
  nodeUpdate : Subsystem
  zLag : Sum
  zLagA : Gain  Gain=ECM.est.lambdaD
  zLagB : Gain  Gain=1-ECM.est.lambdaD
  zLagMem : UnitDelay  SampleTime=-1  HasFrameUpgradeWarning=on
  zLagOld : Switch  Criteria=u2 > Threshold  Threshold=0.5  SaturateOnIntegerOverflow=off  InputSameDT=off
  dTab : Outport
  dCnt : Outport  Port=2
  wires:
  zLag/1 -> zLagMem/1, nodeUpdate/3(z)
  zLagA/1 -> zLag/1
  z/1 -> zLagOld/1, zLagB/1
  first/1 -> TLagOld/2, zLagOld/2
  TLagA/1 -> TLag/1
  zLagB/1 -> zLag/2
  T/1 -> TLagB/1, TLagOld/1
  enable/1 -> nodeUpdate/2(enable)
  TLagOld/1 -> TLagA/1
  zLagOld/1 -> zLagA/1
  TLagB/1 -> TLag/2
  theta/1 -> nodeUpdate/1(theta)
  tab/1 -> nodeUpdate/5(tab)
  TLag/1 -> TLagMem/1, nodeUpdate/4(T)
  cnt/1 -> nodeUpdate/6(cnt)
  zLagMem/1 -> zLagOld/3
  nodeUpdate/1(dTab) -> dTab/1
  nodeUpdate/2(dCnt) -> dCnt/1
  TLagMem/1 -> TLagOld/3

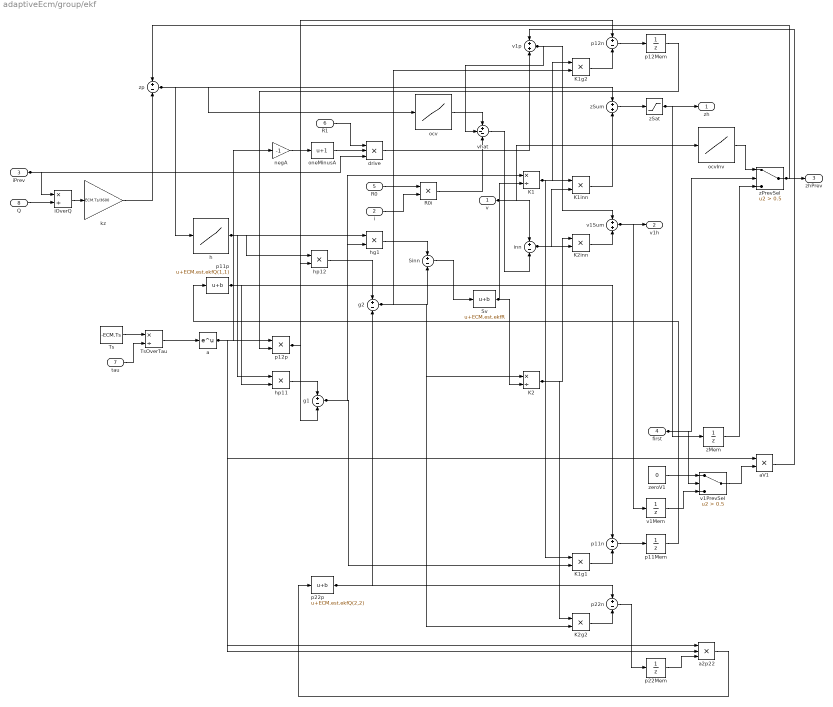
== system adaptiveEcm/group/ekf ==
  v : Inport  PortDimensions=1
  i : Inport  Port=2  PortDimensions=1
  iPrev : Inport  Port=3  PortDimensions=1
  first : Inport  Port=4  PortDimensions=1
  R0 : Inport  Port=5  PortDimensions=1
  R1 : Inport  Port=6  PortDimensions=1
  tau : Inport  Port=7  PortDimensions=1
  Q : Inport  Port=8  PortDimensions=1
  K1 : Product  Inputs=*/
  K1g1 : Product
  K1g2 : Product
  K1inn : Product
  K2 : Product  Inputs=*/
  K2g2 : Product
  K2inn : Product
  R0i : Product
  Sinn : Sum  Inputs=+-
  Sv : Bias  Bias=ECM.est.ekfR  SaturateOnIntegerOverflow=off
  Ts : Constant  Value=-ECM.Ts
  TsOverTau : Product  Inputs=*/
  a : Math
  a2p22 : Product  Inputs=3
  aV1 : Product
  drive : Product  Inputs=3
  g1 : Sum  Inputs=+-
  g2 : Sum  Inputs=+-
  h : Lookup_n-D  NumberOfTableDimensions=1  BreakpointsForDimension1=ECM.est.socBp(1:end-1)  Table=diff(ECM.est.ocv)./diff(ECM.est.socBp)  InterpMethod=Flat  ExtrapMethod=Clip  UseLastTableValue=on  InternalRulePriority=Speed  RndMeth=Simplest
  hg1 : Product
  hp11 : Product
  hp12 : Product
  iOverQ : Product  Inputs=*/
  inn : Sum  Inputs=+-
  kz : Gain  Gain=ECM.Ts/3600
  negA : Gain  Gain=-1
  ocv : Lookup_n-D  NumberOfTableDimensions=1  BreakpointsForDimension1=ECM.est.socBp  Table=ECM.est.ocv  ExtrapMethod=Clip  UseLastTableValue=on  InternalRulePriority=Speed  RndMeth=Simplest
  ocvInv : Lookup_n-D  NumberOfTableDimensions=1  BreakpointsForDimension1=ECM.est.ocv  Table=ECM.est.socBp  ExtrapMethod=Clip  UseLastTableValue=on  InternalRulePriority=Speed  RndMeth=Simplest
  oneMinusA : Bias  Bias=1  SaturateOnIntegerOverflow=off
  p11Mem : UnitDelay  InitialCondition=ECM.est.ekfP0(1,1)  SampleTime=ECM.Ts  HasFrameUpgradeWarning=on
  p11n : Sum  Inputs=+-
  p11p : Bias  Bias=ECM.est.ekfQ(1,1)  SaturateOnIntegerOverflow=off
  p12Mem : UnitDelay  InitialCondition=ECM.est.ekfP0(1,2)  SampleTime=ECM.Ts  HasFrameUpgradeWarning=on
  p12n : Sum  Inputs=+-
  p12p : Product
  p22Mem : UnitDelay  InitialCondition=ECM.est.ekfP0(2,2)  SampleTime=ECM.Ts  HasFrameUpgradeWarning=on
  p22n : Sum  Inputs=+-
  p22p : Bias  Bias=ECM.est.ekfQ(2,2)  SaturateOnIntegerOverflow=off
  v1Mem : UnitDelay  SampleTime=ECM.Ts  HasFrameUpgradeWarning=on
  v1PrevSel : Switch  Criteria=u2 > Threshold  Threshold=0.5  SaturateOnIntegerOverflow=off  InputSameDT=off
  v1Sum : Sum
  v1p : Sum
  vhat : Sum  Inputs=+--
  zMem : UnitDelay  SampleTime=ECM.Ts  HasFrameUpgradeWarning=on
  zPrevSel : Switch  Criteria=u2 > Threshold  Threshold=0.5  SaturateOnIntegerOverflow=off  InputSameDT=off
  zSat : Saturate  UpperLimit=1  LowerLimit=0
  zSum : Sum
  zeroV1 : Constant  Value=0
  zp : Sum  Inputs=+-
  zh : Outport
  v1h : Outport  Port=2
  zhPrev : Outport  Port=3
  wires:
  p22Mem/1 -> a2p22/3
  iPrev/1 -> iOverQ/1, drive/3
  Q/1 -> iOverQ/2
  tau/1 -> TsOverTau/2
  Ts/1 -> TsOverTau/1
  K1inn/1 -> zSum/2
  iOverQ/1 -> kz/1
  kz/1 -> zp/2
  negA/1 -> oneMinusA/1
  zp/1 -> ocv/1, zSum/1, h/1
  zPrevSel/1 -> zp/1, zhPrev/1
  TsOverTau/1 -> a/1
  Sv/1 -> K1/2, K2/2
  h/1 -> hp11/1, hp12/1, hg1/1
  p11p/1 -> p11n/1, hp11/2
  hp11/1 -> g1/1
  a/1 -> a2p22/1, p12p/1, negA/1, a2p22/2, aV1/1
  ocvInv/1 -> zPrevSel/1
  p12p/1 -> g1/2, p12n/1, hp12/2
  p12n/1 -> p12Mem/1
  R1/1 -> drive/1
  R0/1 -> R0i/1
  oneMinusA/1 -> drive/2
  zSat/1 -> zMem/1, zh/1
  hp12/1 -> g2/1
  g1/1 -> K1g1/2, hg1/2, K1/1
  p22p/1 -> g2/2, p22n/1
  drive/1 -> v1p/2
  i/1 -> R0i/2
  K2inn/1 -> v1Sum/2
  hg1/1 -> Sinn/1
  g2/1 -> K1g2/2, K2g2/2, Sinn/2, K2/1
  ocv/1 -> vhat/1
  R0i/1 -> vhat/3
  v1Sum/1 -> v1h/1, v1Mem/1
  Sinn/1 -> Sv/1
  vhat/1 -> inn/2
  first/1 -> zPrevSel/2, v1PrevSel/2
  v/1 -> inn/1, ocvInv/1
  v1p/1 -> vhat/2, v1Sum/1
  K1/1 -> K1g1/1, K1g2/1, K1inn/1
  inn/1 -> K1inn/2, K2inn/2
  K2/1 -> K2inn/1, K2g2/1
  K1g2/1 -> p12n/2
  K1g1/1 -> p11n/2
  v1PrevSel/1 -> aV1/2
  K2g2/1 -> p22n/2
  zSum/1 -> zSat/1
  p11n/1 -> p11Mem/1
  p22n/1 -> p22Mem/1
  p12Mem/1 -> p12p/2
  zeroV1/1 -> v1PrevSel/1
  v1Mem/1 -> v1PrevSel/3
  zMem/1 -> zPrevSel/3
  p11Mem/1 -> p11p/1
  a2p22/1 -> p22p/1
  aV1/1 -> v1p/1

== system adaptiveEcm/group/fill_tabR0 ==
  tab : Inport  PortDimensions=[numel(ECM.est.socBp) numel(ECM.est.tBpC)]
  cnt : Inport  Port=2  PortDimensions=[numel(ECM.est.socBp) numel(ECM.est.tBpC)]
  A : Product
  B2 : Product
  KS : Constant  Value=ECM.est.KS
  KTt : Constant  Value=ECM.est.KT'
  R : Product  Inputs=*/
  Rfill : Product  Inputs=*/
  Rused : Sum
  cConf : Constant  Value=ECM.est.cConfR0
  cntC : Sum
  conf : Product  Inputs=*/
  den : Product  Inputs=3  Multiplication=Matrix(*)
  denE : Bias  Bias=ECM.est.fillEps  SaturateOnIntegerOverflow=off
  filled : Product
  init : Constant  Value=r0Init
  nconf : Gain  Gain=-1
  num : Product  Inputs=3  Multiplication=Matrix(*)
  numE : Bias  Bias=ECM.est.fillEps  SaturateOnIntegerOverflow=off
  omc : Bias  Bias=1  SaturateOnIntegerOverflow=off
  sel : Switch  Criteria=u2 ~= 0  SaturateOnIntegerOverflow=off  InputSameDT=off
  spread : Constant  Value=double(ECM.est.spread)
  used : Outport
  wires:
  den/1 -> denE/1
  R/1 -> A/2
  tab/1 -> R/1, sel/3
  cntC/1 -> conf/2
  cnt/1 -> cntC/1, conf/1
  cConf/1 -> cntC/2
  init/1 -> filled/1, R/2
  conf/1 -> nconf/1, den/2, A/1
  A/1 -> num/2, Rused/1
  KS/1 -> num/1, den/1
  KTt/1 -> num/3, den/3
  nconf/1 -> omc/1
  num/1 -> numE/1
  numE/1 -> Rfill/1
  denE/1 -> Rfill/2
  omc/1 -> B2/1
  Rfill/1 -> B2/2
  B2/1 -> Rused/2
  Rused/1 -> filled/2
  filled/1 -> sel/1
  spread/1 -> sel/2
  sel/1 -> used/1

== system adaptiveEcm/group/fill_tabR1 ==
  tab : Inport  PortDimensions=[numel(ECM.est.socBp) numel(ECM.est.tBpC)]
  cnt : Inport  Port=2  PortDimensions=[numel(ECM.est.socBp) numel(ECM.est.tBpC)]
  A : Product
  B2 : Product
  KS : Constant  Value=ECM.est.KS
  KTt : Constant  Value=ECM.est.KT'
  R : Product  Inputs=*/
  Rfill : Product  Inputs=*/
  Rused : Sum
  cConf : Constant  Value=ECM.est.cConfRc
  cntC : Sum
  conf : Product  Inputs=*/
  den : Product  Inputs=3  Multiplication=Matrix(*)
  denE : Bias  Bias=ECM.est.fillEps  SaturateOnIntegerOverflow=off
  filled : Product
  init : Constant  Value=r1Init
  nconf : Gain  Gain=-1
  num : Product  Inputs=3  Multiplication=Matrix(*)
  numE : Bias  Bias=ECM.est.fillEps  SaturateOnIntegerOverflow=off
  omc : Bias  Bias=1  SaturateOnIntegerOverflow=off
  sel : Switch  Criteria=u2 ~= 0  SaturateOnIntegerOverflow=off  InputSameDT=off
  spread : Constant  Value=double(ECM.est.spread)
  used : Outport
  wires:
  cnt/1 -> cntC/1, conf/1
  cConf/1 -> cntC/2
  cntC/1 -> conf/2
  init/1 -> filled/1, R/2
  tab/1 -> sel/3, R/1
  R/1 -> A/2
  nconf/1 -> omc/1
  conf/1 -> den/2, nconf/1, A/1
  A/1 -> Rused/1, num/2
  KS/1 -> num/1, den/1
  KTt/1 -> num/3, den/3
  num/1 -> numE/1
  den/1 -> denE/1
  spread/1 -> sel/2
  numE/1 -> Rfill/1
  denE/1 -> Rfill/2
  omc/1 -> B2/1
  Rfill/1 -> B2/2
  B2/1 -> Rused/2
  Rused/1 -> filled/2
  filled/1 -> sel/1
  sel/1 -> used/1

== system adaptiveEcm/group/fill_tabTau ==
  tab : Inport  PortDimensions=[numel(ECM.est.socBp) numel(ECM.est.tBpC)]
  cnt : Inport  Port=2  PortDimensions=[numel(ECM.est.socBp) numel(ECM.est.tBpC)]
  A : Product
  B2 : Product
  KS : Constant  Value=ECM.est.KS
  KTt : Constant  Value=ECM.est.KT'
  R : Product  Inputs=*/
  Rfill : Product  Inputs=*/
  Rused : Sum
  cConf : Constant  Value=ECM.est.cConfRc
  cntC : Sum
  conf : Product  Inputs=*/
  den : Product  Inputs=3  Multiplication=Matrix(*)
  denE : Bias  Bias=ECM.est.fillEps  SaturateOnIntegerOverflow=off
  filled : Product
  init : Constant  Value=tauInit
  nconf : Gain  Gain=-1
  num : Product  Inputs=3  Multiplication=Matrix(*)
  numE : Bias  Bias=ECM.est.fillEps  SaturateOnIntegerOverflow=off
  omc : Bias  Bias=1  SaturateOnIntegerOverflow=off
  sel : Switch  Criteria=u2 ~= 0  SaturateOnIntegerOverflow=off  InputSameDT=off
  spread : Constant  Value=double(ECM.est.spread)
  used : Outport
  wires:
  cntC/1 -> conf/2
  cnt/1 -> cntC/1, conf/1
  R/1 -> A/2
  cConf/1 -> cntC/2
  omc/1 -> B2/1
  init/1 -> R/2, filled/1
  tab/1 -> sel/3, R/1
  conf/1 -> den/2, nconf/1, A/1
  A/1 -> num/2, Rused/1
  KS/1 -> num/1, den/1
  KTt/1 -> num/3, den/3
  nconf/1 -> omc/1
  num/1 -> numE/1
  filled/1 -> sel/1
  denE/1 -> Rfill/2
  den/1 -> denE/1
  Rused/1 -> filled/2
  numE/1 -> Rfill/1
  Rfill/1 -> B2/2
  B2/1 -> Rused/2
  spread/1 -> sel/2
  sel/1 -> used/1

== system adaptiveEcm/group/opPoint ==
  z : Inport  PortDimensions=1
  T : Inport  Port=2  PortDimensions=1
  tabR0 : Inport  Port=3  PortDimensions=[numel(ECM.est.socBp) numel(ECM.est.tBpC)]
  tabR1 : Inport  Port=4  PortDimensions=[numel(ECM.est.socBp) numel(ECM.est.tBpC)]
  tabTau : Inport  Port=5  PortDimensions=[numel(ECM.est.socBp) numel(ECM.est.tBpC)]
  interpR0 : Interpolation_n-D  TableSource=Input port  InternalRulePriority=Speed
      settings: InputPortMap=u0,u1,u2,u3,p2
  interpR1 : Interpolation_n-D  TableSource=Input port  InternalRulePriority=Speed
      settings: InputPortMap=u0,u1,u2,u3,p2
  interptau : Interpolation_n-D  TableSource=Input port  InternalRulePriority=Speed
      settings: InputPortMap=u0,u1,u2,u3,p2
  preT : PreLookup  BreakpointsData=ECM.est.tBpC
  preZ : PreLookup  BreakpointsData=ECM.est.socBp
  R0 : Outport
  R1 : Outport  Port=2
  tau : Outport  Port=3
  wires:
  tabR0/1 -> interpR0/5
  tabR1/1 -> interpR1/5
  z/1 -> preZ/1
  tabTau/1 -> interptau/5
  T/1 -> preT/1
  preZ/1 -> interpR0/1, interpR1/1, interptau/1
  preZ/2 -> interpR0/2, interpR1/2, interptau/2
  preT/1 -> interpR0/3, interpR1/3, interptau/3
  preT/2 -> interpR0/4, interpR1/4, interptau/4
  interpR0/1 -> R0/1
  interptau/1 -> tau/1
  interpR1/1 -> R1/1

== system adaptiveEcm/group/r0Ident ==
  v : Inport  PortDimensions=1
  vPrev : Inport  Port=2  PortDimensions=1
  i : Inport  Port=3  PortDimensions=1
  iPrev : Inport  Port=4  PortDimensions=1
  first : Inport  Port=5  PortDimensions=1
  K : Product  Inputs=*/
  Ke : Product
  KphiP : Product
  den : Bias  Bias=ECM.est.lambda0  SaturateOnIntegerOverflow=off
  di : Sum  Inputs=+-
  dv : Sum  Inputs=+-
  e : Sum  Inputs=+-
  inf : RelationalOperator  Operator=<  OutDataTypeStr=boolean  RndMeth=Simplest  InputSameDT=off
  info : Constant  Value=ECM.est.infoR0
  pCap : MinMax  Inputs=2
  pDiv : Gain  Gain=1/ECM.est.lambda0
  pMax : Constant  Value=ECM.est.pMaxR0
  pMem : UnitDelay  InitialCondition=ECM.est.p0R0  SampleTime=ECM.Ts  HasFrameUpgradeWarning=on
  pNum : Sum  Inputs=+-
  pPhi : Product
  phi : Gain  Gain=-1
  phiPphi : Product
  phiSel : Switch  Criteria=u2 > Threshold  Threshold=0.5  SaturateOnIntegerOverflow=off  InputSameDT=off
  phiTh : Product
  th : Sum
  thMem : UnitDelay  InitialCondition=th0Init  SampleTime=ECM.Ts  HasFrameUpgradeWarning=on
  zeroPhi : Constant  Value=0
  R0 : Outport
  informed : Outport  Port=2
  wires:
  di/1 -> phi/1
  i/1 -> di/1
  phiSel/1 -> pPhi/2, phiTh/1, phiPphi/2
  phi/1 -> phiSel/3
  iPrev/1 -> di/2
  zeroPhi/1 -> phiSel/1
  KphiP/1 -> pNum/2
  first/1 -> phiSel/2
  dv/1 -> e/1
  v/1 -> dv/1
  vPrev/1 -> dv/2
  thMem/1 -> th/1, phiTh/2
  phiPphi/1 -> den/1
  phiTh/1 -> e/2
  info/1 -> inf/2
  pCap/1 -> pMem/1, inf/1
  den/1 -> K/2
  pPhi/1 -> phiPphi/1, KphiP/2, K/1
  e/1 -> Ke/2
  pNum/1 -> pDiv/1
  K/1 -> Ke/1, KphiP/1
  Ke/1 -> th/2
  th/1 -> R0/1, thMem/1
  inf/1 -> informed/1
  pDiv/1 -> pCap/1
  pMax/1 -> pCap/2
  pMem/1 -> pPhi/1, pNum/1

== system adaptiveEcm/group/r0Table ==
  theta : Inport  PortDimensions=1
  enable : Inport  Port=2  PortDimensions=1
  z : Inport  Port=3  PortDimensions=1
  T : Inport  Port=4  PortDimensions=1
  first : Inport  Port=5  PortDimensions=1
  tab : Inport  Port=6  PortDimensions=[numel(ECM.est.socBp) numel(ECM.est.tBpC)]
  cnt : Inport  Port=7  PortDimensions=[numel(ECM.est.socBp) numel(ECM.est.tBpC)]
  TLag : Sum
  TLagA : Gain  Gain=ECM.est.lambda0
  TLagB : Gain  Gain=1-ECM.est.lambda0
  TLagMem : UnitDelay  SampleTime=-1  HasFrameUpgradeWarning=on
  TLagOld : Switch  Criteria=u2 > Threshold  Threshold=0.5  SaturateOnIntegerOverflow=off  InputSameDT=off
  nodeUpdate : Subsystem
  zLag : Sum
  zLagA : Gain  Gain=ECM.est.lambda0
  zLagB : Gain  Gain=1-ECM.est.lambda0
  zLagMem : UnitDelay  SampleTime=-1  HasFrameUpgradeWarning=on
  zLagOld : Switch  Criteria=u2 > Threshold  Threshold=0.5  SaturateOnIntegerOverflow=off  InputSameDT=off
  dTab : Outport
  dCnt : Outport  Port=2
  wires:
  z/1 -> zLagB/1, zLagOld/1
  zLagB/1 -> zLag/2
  first/1 -> zLagOld/2, TLagOld/2
  T/1 -> TLagOld/1, TLagB/1
  TLagOld/1 -> TLagA/1
  zLagOld/1 -> zLagA/1
  TLagMem/1 -> TLagOld/3
  zLagA/1 -> zLag/1
  TLagB/1 -> TLag/2
  TLagA/1 -> TLag/1
  theta/1 -> nodeUpdate/1(theta)
  cnt/1 -> nodeUpdate/6(cnt)
  zLag/1 -> zLagMem/1, nodeUpdate/3(z)
  enable/1 -> nodeUpdate/2(enable)
  tab/1 -> nodeUpdate/5(tab)
  nodeUpdate/2(dCnt) -> dCnt/1
  TLag/1 -> TLagMem/1, nodeUpdate/4(T)
  zLagMem/1 -> zLagOld/3
  nodeUpdate/1(dTab) -> dTab/1

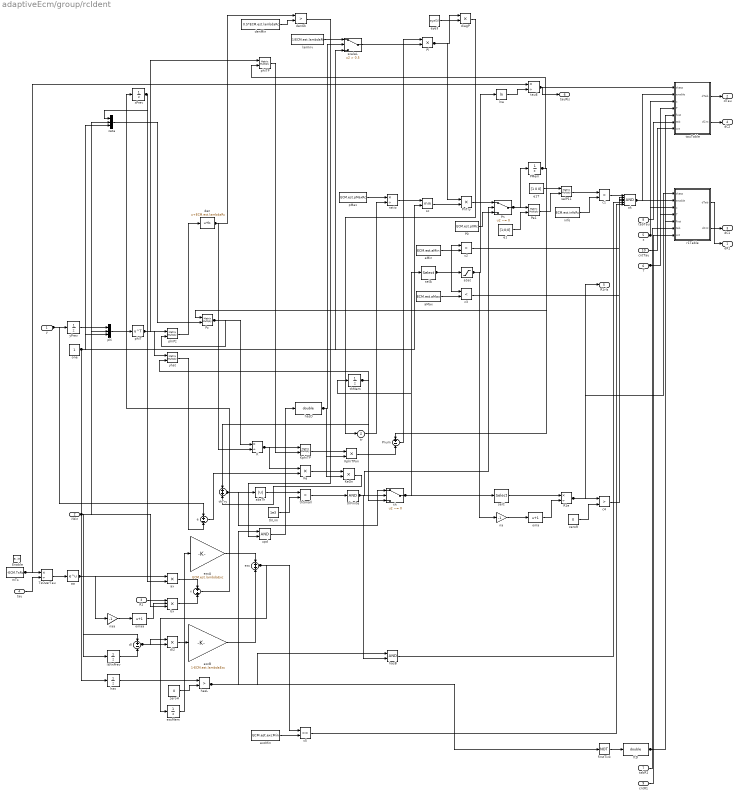
== system adaptiveEcm/group/rcIdent ==
  y : Inport  PortDimensions=1
  iWin : Inport  Port=2  PortDimensions=1
  R1 : Inport  Port=3  PortDimensions=1
  tau : Inport  Port=4  PortDimensions=1
  z : Inport  Port=5  PortDimensions=1
  T : Inport  Port=6  PortDimensions=1
  tabR1 : Inport  Port=7  PortDimensions=[numel(ECM.est.socBp) numel(ECM.est.tBpC)]
  tabTau : Inport  Port=8  PortDimensions=[numel(ECM.est.socBp) numel(ECM.est.tBpC)]
  cntR1 : Inport  Port=9  PortDimensions=[numel(ECM.est.socBp) numel(ECM.est.tBpC)]
  cntTau : Inport  Port=10  PortDimensions=[numel(ECM.est.socBp) numel(ECM.est.tBpC)]
  Enable : EnablePort
  K : Product  Inputs=*/
  Ke : Product
  KeOn : Product
  KphiTP : Product  Multiplication=Matrix(*)
  KphiTPon : Product
  P0 : Constant  Value=ECM.est.p0Rc
  PMem : UnitDelay  InitialCondition=ECM.est.p0Rc  SampleTime=-1  HasFrameUpgradeWarning=on
  Pe1 : Product  Multiplication=Matrix(*)
  Pl : Product
  Pn : Switch  Criteria=u2 ~= 0  SaturateOnIntegerOverflow=off  InputSameDT=off
  PnTry : Product
  Pnum : Sum  Inputs=+-
  Pz : Product  Multiplication=Matrix(*)
  R1e : Product  Inputs=*/
  TsOverTau : Product  Inputs=*/
  aMax : Constant  Value=ECM.est.aMax
  aMin : Constant  Value=ECM.est.aMin
  aSat : Saturate  UpperLimit=ECM.est.aMax  LowerLimit=ECM.est.aMin
  aa : Math
  absTh : Abs  SaturateOnIntegerOverflow=off
  ax : Product
  bx : Product  Inputs=3
  c1 : RelationalOperator  Operator=<  OutDataTypeStr=boolean  RndMeth=Simplest  InputSameDT=off
  c2 : RelationalOperator  Operator=>  OutDataTypeStr=boolean  RndMeth=Simplest  InputSameDT=off
  c3 : RelationalOperator  Operator=<  OutDataTypeStr=boolean  RndMeth=Simplest  InputSameDT=off
  c4 : RelationalOperator  Operator=>  OutDataTypeStr=boolean  RndMeth=Simplest  InputSameDT=off
  c5 : RelationalOperator  OutDataTypeStr=boolean  RndMeth=Simplest  InputSameDT=off
  dI : Sum  Inputs=+-
  dI2 : Product
  den : Bias  Bias=ECM.est.lambdaRc  SaturateOnIntegerOverflow=off
  denMin : Constant  Value=0.5*ECM.est.lambdaRc
  denOk : RelationalOperator  Operator=>  OutDataTypeStr=boolean  RndMeth=Simplest  InputSameDT=off
  diagP : Product
  e : Sum  Inputs=+-
  e1 : Constant  Value=[1;0;0]  VectorParams1D=off
  e1T : Constant  Value=[1 0 0]  VectorParams1D=off
  exc : Sum
  excA : Gain  Gain=ECM.est.lambdaExc
  excB : Gain  Gain=1-ECM.est.lambdaExc
  excMem : UnitDelay  SampleTime=-1  HasFrameUpgradeWarning=on
  excMin : Constant  Value=ECM.est.excMin
  eye3 : Constant  Value=eye(3)
  firstTick : Logic  Operator=NOT  AllPortsSameDT=off  OutDataTypeStr=boolean
  ftD : DataTypeConversion  OutDataTypeStr=double  SaturateOnIntegerOverflow=off  RndMeth=Floor
  has : UnitDelay  SampleTime=-1  HasFrameUpgradeWarning=on
  hasB : Logic  AllPortsSameDT=off  OutDataTypeStr=boolean
  hasD : DataTypeConversion  OutDataTypeStr=double  SaturateOnIntegerOverflow=off  RndMeth=Floor
  hasL : RelationalOperator  Operator=>  OutDataTypeStr=boolean  RndMeth=Simplest  InputSameDT=off
  iWinPrev : UnitDelay  SampleTime=-1  HasFrameUpgradeWarning=on
  info : Constant  Value=ECM.est.infoRc
  lamInv : Constant  Value=1/ECM.est.lambdaRc
  lna : Math  Operator=log
  mTs : Constant  Value=-ECM.TsRc
  na : Gain  Gain=-1
  naa : Gain  Gain=-1
  ok : Logic  Inputs=6  AllPortsSameDT=off  OutDataTypeStr=boolean
  oma : Bias  Bias=1  SaturateOnIntegerOverflow=off
  omaa : Bias  Bias=1  SaturateOnIntegerOverflow=off
  one : Constant
  pMax : Constant  Value=ECM.est.pMaxRc
  phi : Concatenate  NumInputs=3  Mode=Multidimensional array
  phiPz : Product  Multiplication=Matrix(*)
  phiT : Math  Operator=transpose
  phiTP : Product  Multiplication=Matrix(*)
  r1Table : Subsystem
  ratio : Product  Inputs=*/
  sc : MinMax  Inputs=2
  scaleL : Switch  Criteria=u2 > Threshold  Threshold=0.5  SaturateOnIntegerOverflow=off  InputSameDT=off
  selA : Selector  InputPortWidth=3  IndexOptions=Index vector (dialog)  Indices=1  OutputSizes=1
  selC : Selector  InputPortWidth=3  IndexOptions=Index vector (dialog)  Indices=2  OutputSizes=1
  selP11 : Product  Multiplication=Matrix(*)
  tauE : Product  Inputs=*/
  tauTable : Subsystem
  th : Switch  Criteria=u2 ~= 0  SaturateOnIntegerOverflow=off  InputSameDT=off
  thFinite : Logic  Inputs=1  AllPortsSameDT=off  OutDataTypeStr=boolean
  thLim : Constant  Value=1e3
  thMem : UnitDelay  InitialCondition=thRcInit  SampleTime=-1  HasFrameUpgradeWarning=on
  thSmall : RelationalOperator  Operator=<  OutDataTypeStr=boolean  RndMeth=Simplest  InputSameDT=off
  thTry : Sum
  tr : Sum  Inputs=+
  upd : Logic  AllPortsSameDT=off  OutDataTypeStr=boolean
  x : Sum
  xPrev : UnitDelay  SampleTime=-1  HasFrameUpgradeWarning=on
  yPrev : UnitDelay  SampleTime=-1  HasFrameUpgradeWarning=on
  yhat : Product  Multiplication=Matrix(*)
  zeroH : Constant  Value=0
  zeroR : Constant  Value=0
  zeta : Concatenate  NumInputs=3  Mode=Multidimensional array
  dR1 : Outport  OutputWhenDisabled=reset  InitialOutput=0
  dTau : Outport  Port=2  OutputWhenDisabled=reset  InitialOutput=0
  dC1 : Outport  Port=3  OutputWhenDisabled=reset  InitialOutput=0
  dC2 : Outport  Port=4  OutputWhenDisabled=reset  InitialOutput=0
  R1rls : Outport  Port=5  InitialOutput=0
  tauRls : Outport  Port=6  InitialOutput=0
  wires:
  mTs/1 -> tauE/1, TsOverTau/1
  den/1 -> denOk/1, K/2
  tau/1 -> TsOverTau/2
  y/1 -> e/1, yPrev/1
  yPrev/1 -> phi/1
  TsOverTau/1 -> aa/1
  aa/1 -> ax/1, naa/1
  KeOn/1 -> thTry/2
  one/1 -> has/1, zeta/3, scaleL/3, phi/3, sc/2
  iWin/1 -> bx/3, zeta/2, phi/2, iWinPrev/1, dI/1
  zeta/1 -> Pz/2
  iWinPrev/1 -> dI/2
  phi/1 -> phiT/1
  Pl/1 -> diagP/1, PnTry/1
  naa/1 -> omaa/1
  th/1 -> thMem/1, selA/1, selC/1
  thTry/1 -> th/1, absTh/1
  has/1 -> hasL/1
  tauTable/2(dCnt) -> dC2/1
  xPrev/1 -> zeta/1, ax/2
  ax/1 -> x/1
  phiPz/1 -> den/1
  phiT/1 -> phiTP/1, phiPz/1, yhat/1
  R1/1 -> bx/1
  omaa/1 -> bx/2
  thLim/1 -> thSmall/2
  dI/1 -> dI2/1, dI2/2
  yhat/1 -> e/2
  KphiTP/1 -> KphiTPon/1
  bx/1 -> x/2
  excA/1 -> exc/1
  thMem/1 -> yhat/2, thTry/1, th/3
  pMax/1 -> ratio/1
  c3/1 -> ok/3
  dI2/1 -> excB/1
  KphiTPon/1 -> Pnum/2
  zeroH/1 -> hasL/2
  scaleL/1 -> Pl/2
  excMem/1 -> excA/1
  e/1 -> Ke/2
  tauTable/1(dTab) -> dTau/1
  exc/1 -> excMem/1, c5/1
  c5/1 -> ok/6
  hasD/1 -> KeOn/2, KphiTPon/2, scaleL/2
  x/1 -> xPrev/1
  Pz/1 -> phiPz/2, K/1
  excB/1 -> exc/2
  hasL/1 -> hasB/1, upd/1, firstTick/1
  denMin/1 -> denOk/2
  phiTP/1 -> KphiTP/2
  tauE/1 -> tauTable/1(theta), tauRls/1
  K/1 -> Ke/1, KphiTP/1
  Ke/1 -> KeOn/1
  absTh/1 -> thSmall/1
  upd/1 -> hasD/1
  thFinite/1 -> Pn/2, th/2, hasB/2
  excMin/1 -> c5/2
  denOk/1 -> upd/2
  lamInv/1 -> scaleL/1
  info/1 -> c1/2
  thSmall/1 -> thFinite/1
  selA/1 -> c2/1, aSat/1, c3/1
  tr/1 -> ratio/2
  ratio/1 -> sc/1
  aMin/1 -> c2/2
  diagP/1 -> tr/1
  Pnum/1 -> Pl/1
  hasB/1 -> ok/5
  eye3/1 -> diagP/2
  Pn/1 -> PMem/1, Pe1/1
  sc/1 -> PnTry/2
  aMax/1 -> c3/2
  PnTry/1 -> Pn/1
  P0/1 -> Pn/3
  c2/1 -> ok/2
  aSat/1 -> na/1, lna/1
  lna/1 -> tauE/2
  oma/1 -> R1e/2
  e1/1 -> Pe1/2
  selC/1 -> R1e/1
  na/1 -> oma/1
  PMem/1 -> phiTP/2, Pnum/1, Pz/1
  e1T/1 -> selP11/1
  Pe1/1 -> selP11/2
  selP11/1 -> c1/1
  R1e/1 -> r1Table/1(theta), R1rls/1, c4/1
  zeroR/1 -> c4/2
  c1/1 -> ok/1
  c4/1 -> ok/4
  firstTick/1 -> ftD/1
  ok/1 -> r1Table/2(enable), tauTable/2(enable)
  tabTau/1 -> tauTable/6(tab)
  z/1 -> r1Table/3(z), tauTable/3(z)
  cntTau/1 -> tauTable/7(cnt)
  T/1 -> r1Table/4(T), tauTable/4(T)
  ftD/1 -> r1Table/5(first), tauTable/5(first)
  tabR1/1 -> r1Table/6(tab)
  cntR1/1 -> r1Table/7(cnt)
  r1Table/1(dTab) -> dR1/1
  r1Table/2(dCnt) -> dC1/1
